simulink model "Balancing_Robot_Nom_Tracking_Quanser"  (R2024b)
settings: Solver=ode23  StartTime=0.0  StopTime=30  RelTol=1e-3
undefined symbols (not defined in the file): C_filter, drv, dspblkCoreblockFVToolHelper, gbox, gcbh, K_Nom_LQR_Br, Nu, Nx, sens, T, wheel
settings Model: Creator=liliy  LastModifiedBy=liliy

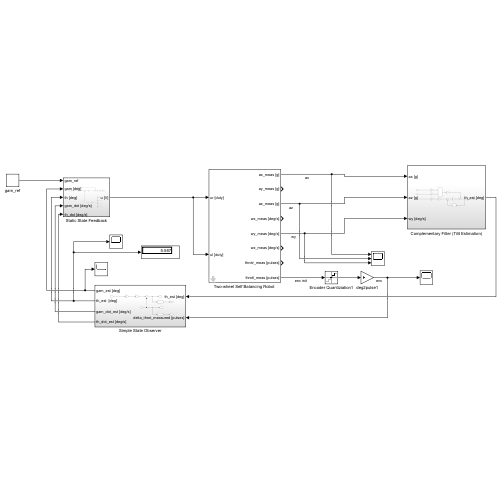
[thumbnail: Simulink's stored preview of the top-level diagram]
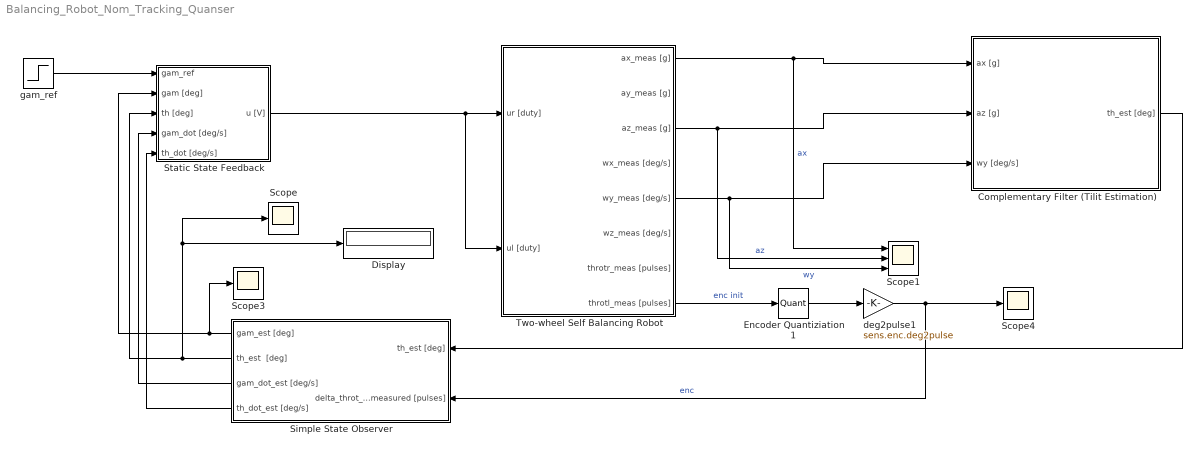
== system Balancing_Robot_Nom_Tracking_Quanser ==
  Complementary Filter (Tilit Estimation) : Subsystem
  Display : Display
  Encoder Quantiziation1 : Quantizer  QuantizationInterval=sens.enc.pulse2deg
  Scope : Scope
  Scope1 : Scope  NumInputPorts=3
  Scope3 : Scope
  Scope4 : Scope
  Simple State Observer : Subsystem
  Static State Feedback : Subsystem
  "Two-wheel Self Balancing Robot " : Subsystem  mask(Balancing robot (longitudinal + lateral dynamics)){initState=[0, 0, 0, 0, 0, 0], Ts=T}
      mask prompts: initState "Initial state [gam(0), psi(0), th(0), dot_gam(0), dot_psi(0), dot_th(0)]'"; Ts "Sample time:"
      mask help:
      | Balancing robot dynamic model.
      | Includes both the longitudinal and lateral (yaw) dynamics.
      mask init:
      | %% General parameters and conversion gains
      | 
      | %   gravity acc [m/s^2]
      | g = 9.81;
      | 
      | %   conversion gains
      | rpm2rads = 2*pi/60;         %   [rpm]   -> [rad/s]
      | rads2rpm = 60/2/pi;         %   [rad/s] -> [rpm]
      | rpm2degs = 360/60;          %   [rpm]   -> [deg/s]
      | degs2rpm = 60/360;          %   [deg/s] -> [rpm]
      | deg2rad = pi/180;           %   [deg]   -> [rad]
      | rad2deg = 180/pi;           %   [rad]   -> [deg]
      | g2ms2 = g;                  %   [acc_g] -> [m/s^2]
      | ms22g = 1/g;                %   [m/s^2] -> [acc_g]
      | ozin2Nm = 0.706e-2;         %   [oz*inch] -> [N*m]
      | 
      | 
      | %%  Battery data
      | 
      | %   electrical data
      | batt.UN = 11.1;     %   nominal voltage
      | 
      | 
      | %%  H-bridge PWM voltage driver
      | 
      | drv.Vbus = batt.UN;                     %   H-bridge DC bus voltage  
      | drv.pwm.bits = 8;                       %   PWM resolution [bits]
      | drv.pwm.levels = 2^drv.pwm.bits;        %   PWM levels
      | drv.pwm.Fs = 490;                       %   PWM frequency
      | drv.dutymax = drv.pwm.levels-1;         %   max duty cycle code
      | drv.duty2V = drv.Vbus/drv.dutymax;      %   duty cycle code (0-255) to voltage
      | drv.V2duty = drv.dutymax/drv.Vbus;      %   voltage to duty cycle code (0-255)
      | 
      | 
      | %%  Gearbox data 
      | 
      | gbox.N = 30;            %   reduction ratio
      | 
      | 
      | %%  Sensors data - Hall-effect encoder
      | 
      | %   Hall-effect encoder
      | sens.enc.ppr = 16*4;    %   pulses per rotation at motor side (w/ quadrature decoding)
      | sens.enc.pulse2deg = 360/sens.enc.ppr;
      | sens.enc.pulse2rad = 2*pi/sens.enc.ppr;
      | sens.enc.deg2pulse = sens.enc.ppr/360;
      | sens.enc.rad2pulse = sens.enc.ppr/2/pi;
      | 
      | 
      | %%  Sensors data - MPU6050 (accelerometer + gyro)
      | 
      | %   center of mass (CoM) position
      | sens.mpu.xb = 0;
      | sens.mpu.yb = 0;
      | sens.mpu.zb = 13.5e-3;
      | 
      | %       MPU6050 embedded accelerometer specs
      | sens.mpu.acc.bits = 16;
      | sens.mpu.acc.fs_g = 16;                                                         %   full-scale in "g" units
      | sens.mpu.acc.fs = sens.mpu.acc.fs_g * g2ms2;                                    %   full-scale in [m/s^2] 
      | sens.mpu.acc.g2LSB = floor(2^(sens.mpu.acc.bits-1)/sens.mpu.acc.fs_g);          %   sensitivity [LSB/g]
      | sens.mpu.acc.ms22LSB = sens.mpu.acc.g2LSB * ms22g;                              %   sensitvity [LSB/(m/s^2)]
      | sens.mpu.acc.LSB2g = sens.mpu.acc.fs_g/2^(sens.mpu.acc.bits-1);                 %   output quantization step [g/LSB]
      | sens.mpu.acc.LSB2ms2 = sens.mpu.acc.LSB2g * g2ms2;                              %   output quantization step [ms2/LSB]
      | sens.mpu.acc.bw = 94;                                                           %   output low-pass filter bandwidth
      | sens.mpu.acc.noisestd = 400e-6*sqrt(100);                                       %   output noise std [g-rms]
      | sens.mpu.acc.noisevar = sens.mpu.acc.noisestd^2;                                %   output noise var [g^2]
      | 
      | %       MPU6050 embdedded gyroscope specs
      | sens.mpu.gyro.bits = 16;
      | sens.mpu.gyro.fs_degs = 250;                                                    %   full scale in [deg/s (dps)]
      | sens.mpu.gyro.fs = sens.mpu.gyro.fs_degs * deg2rad;                             %   full scale in [rad/s]
      | sens.mpu.gyro.degs2LSB = floor(2^(sens.mpu.gyro.bits-1)/sens.mpu.gyro.fs_degs);	%   sensitivity [LSB/degs]
      | sens.mpu.gyro.rads2LSB = sens.mpu.gyro.degs2LSB * rad2deg;                      %   sensitivity [LSB/rads] 
      | sens.mpu.gyro.LSB2degs = sens.mpu.gyro.fs_degs/2^(sens.mpu.gyro.bits-1);        %   output quantization step [degs/LSB]
      | sens.mpu.gyro.LSB2rads = sens.mpu.gyro.LSB2degs * deg2rad;                      %   output quantization step [rads/LSB]
      | sens.mpu.gyro.bw = 98;                                                          %   output low-pass filter bandwidth
      | sens.mpu.gyro.noisestd = 5e-3*sqrt(100);                                        %   output noise std [degs-rms]
      | sens.mpu.gyro.noisevar = sens.mpu.acc.noisestd ^2;                              %   output noise var [degs^2]
      mask Help:
      | Riccardo Antonello (antonello@dei.unipd.it)
      | 
      | May 19, 2020
      | 
      | Dept. of Information Engineering, University of Padova
  deg2pulse1 : Gain  Gain=sens.enc.deg2pulse
  gam_ref : Step  Time=0  After=0.1/wheel.r*rad2deg  SampleTime=0
  wires:
  "Two-wheel Self Balancing Robot "/1(ax_meas [g]) -> Scope1/1, Complementary Filter (Tilit Estimation)/1(ax [g])  "ax"
  "Two-wheel Self Balancing Robot "/3(az_meas [g]) -> Scope1/2, Complementary Filter (Tilit Estimation)/2(az [g])  "az"
  "Two-wheel Self Balancing Robot "/5(wy_meas [deg/s]) -> Scope1/3, Complementary Filter (Tilit Estimation)/3(wy [deg/s])  "wy"
  Complementary Filter (Tilit Estimation)/1(th_est [deg]) -> Simple State Observer/1(th_est [deg])
  Simple State Observer/1(gam_est [deg]) -> Scope3/1, Static State Feedback/2(gam [deg])
  Simple State Observer/2(th_est  [deg]) -> Scope/1, Display/1, Static State Feedback/3(th [deg])
  Simple State Observer/3(gam_dot_est [deg/s]) -> Static State Feedback/4(gam_dot [deg/s])
  Simple State Observer/4(th_dot_est [deg/s]) -> Static State Feedback/5(th_dot [deg/s])
  gam_ref/1 -> Static State Feedback/1(gam_ref)
  Static State Feedback/1(u [V]) -> "Two-wheel Self Balancing Robot "/2(ul [duty]), "Two-wheel Self Balancing Robot "/1(ur [duty])
  Encoder Quantiziation1/1 -> deg2pulse1/1
  "Two-wheel Self Balancing Robot "/8(throtl_meas [pulses]) -> Encoder Quantiziation1/1  "enc init"
  deg2pulse1/1 -> Scope4/1, Simple State Observer/2(delta_throt_measured [pulses])  "enc"

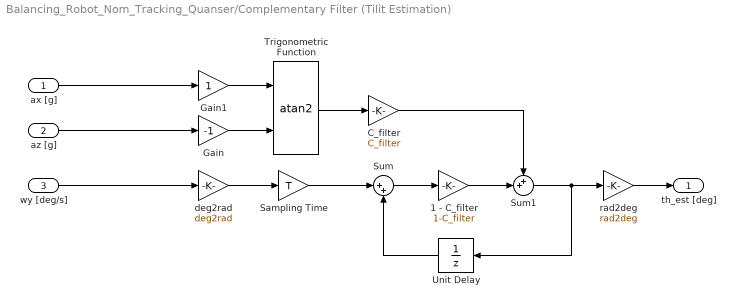
== system Balancing_Robot_Nom_Tracking_Quanser/Complementary Filter (Tilit Estimation) ==
  ax [g] : Inport
  az [g] : Inport  Port=2
  wy [deg/s] : Inport  Port=3
  1 - C_filter : Gain  Gain=1-C_filter
  C_filter : Gain  Gain=C_filter
  Gain : Gain  Gain=-1
  Gain1 : Gain
  Sampling Time : Gain  Gain=T
  Sum : Sum  Inputs=|++
  Sum1 : Sum  Inputs=++|
  Trigonometric Function : Trigonometry  Operator=atan2
  Unit Delay : UnitDelay  SampleTime=T  HasFrameUpgradeWarning=on
  deg2rad : Gain  Gain=deg2rad
  rad2deg : Gain  Gain=rad2deg
  th_est [deg] : Outport
  wires:
  Trigonometric Function/1 -> C_filter/1
  Gain/1 -> Trigonometric Function/2
  rad2deg/1 -> th_est [deg]/1
  deg2rad/1 -> Sampling Time/1
  Sum/1 -> 1 - C_filter/1
  Gain1/1 -> Trigonometric Function/1
  Sum1/1 -> Unit Delay/1, rad2deg/1
  Sampling Time/1 -> Sum/1
  1 - C_filter/1 -> Sum1/2
  Unit Delay/1 -> Sum/2
  C_filter/1 -> Sum1/1
  ax [g]/1 -> Gain1/1
  az [g]/1 -> Gain/1
  wy [deg/s]/1 -> deg2rad/1

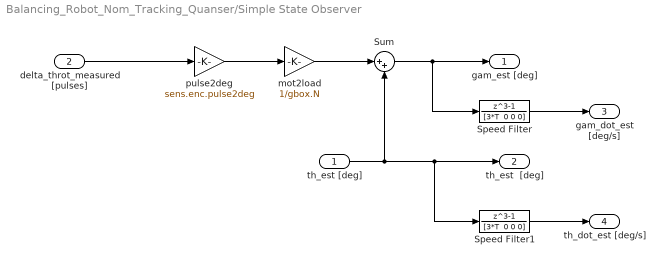
== system Balancing_Robot_Nom_Tracking_Quanser/Simple State Observer ==
  th_est [deg] : Inport
  delta_throt_measured [pulses] : Inport  Port=2
  Speed Filter : DiscreteTransferFcn  LoadFcn=dspblkCoreblockFVToolHelper(gcbh,'load');  Numerator=[1 0 0 -1]  Denominator="[3*T  0 0 0]"
      settings: CopyFcn=dspblkCoreblockFVToolHelper(gcbh,'copy');  DeleteFcn=dspblkCoreblockFVToolHelper(gcbh,'close');  ModelCloseFcn=dspblkCoreblockFVToolHelper(gcbh,'close');  PreSaveFcn=dspblkCoreblockFVToolHelper(gcbh,'presave');  PostSaveFcn=dspblkCoreblockFVToolHelper(gcbh,'postsave');  CloseFcn=dspblkCoreblockFVToolHelper(gcbh,'close');
  Speed Filter1 : DiscreteTransferFcn  LoadFcn=dspblkCoreblockFVToolHelper(gcbh,'load');  Numerator=[1 0 0 -1]  Denominator="[3*T  0 0 0]"
      settings: CopyFcn=dspblkCoreblockFVToolHelper(gcbh,'copy');  DeleteFcn=dspblkCoreblockFVToolHelper(gcbh,'close');  ModelCloseFcn=dspblkCoreblockFVToolHelper(gcbh,'close');  PreSaveFcn=dspblkCoreblockFVToolHelper(gcbh,'presave');  PostSaveFcn=dspblkCoreblockFVToolHelper(gcbh,'postsave');  CloseFcn=dspblkCoreblockFVToolHelper(gcbh,'close');
  Sum : Sum  Inputs=|++
  mot2load : Gain  Gain=1/gbox.N
  pulse2deg : Gain  Gain=sens.enc.pulse2deg
  gam_est [deg] : Outport
  th_est  [deg] : Outport  Port=2
  gam_dot_est [deg/s] : Outport  Port=3
  th_dot_est [deg/s] : Outport  Port=4
  wires:
  Sum/1 -> Speed Filter/1, gam_est [deg]/1
  pulse2deg/1 -> mot2load/1
  Speed Filter/1 -> gam_dot_est [deg/s]/1
  delta_throt_measured [pulses]/1 -> pulse2deg/1
  Speed Filter1/1 -> th_dot_est [deg/s]/1
  th_est [deg]/1 -> Sum/2, Speed Filter1/1, th_est  [deg]/1
  mot2load/1 -> Sum/1

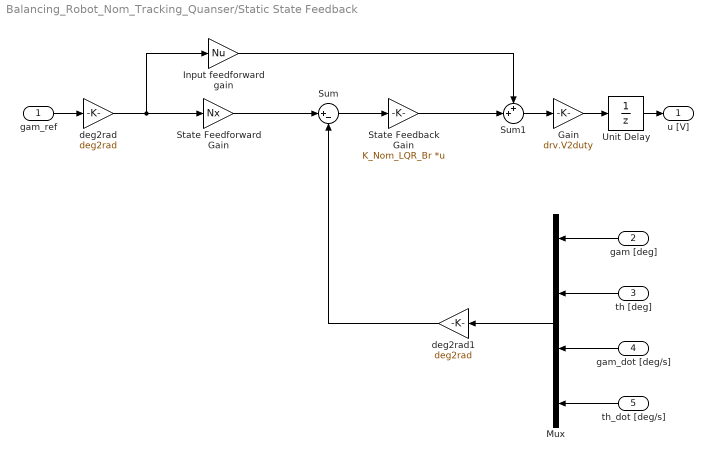
== system Balancing_Robot_Nom_Tracking_Quanser/Static State Feedback ==
  gam_ref : Inport
  gam [deg] : Inport  Port=2
  th [deg] : Inport  Port=3
  gam_dot [deg/s] : Inport  Port=4
  th_dot [deg/s] : Inport  Port=5
  Gain : Gain  Gain=drv.V2duty
  Input feedforward gain : Gain  Gain=Nu
  Mux : Mux
  State Feedback Gain : Gain  Gain=K_Nom_LQR_Br  Multiplication=Matrix(K*u)
  State Feedforward Gain : Gain  Gain=Nx
  Sum : Sum  Inputs=|+-
  Sum1 : Sum  Inputs=++|
  Unit Delay : UnitDelay  SampleTime=T  HasFrameUpgradeWarning=on
  deg2rad : Gain  Gain=deg2rad
  deg2rad1 : Gain  Gain=deg2rad
  u [V] : Outport
  wires:
  gam_ref/1 -> deg2rad/1
  deg2rad/1 -> Input feedforward gain/1, State Feedforward Gain/1
  State Feedforward Gain/1 -> Sum/1
  Sum/1 -> State Feedback Gain/1
  State Feedback Gain/1 -> Sum1/2
  Input feedforward gain/1 -> Sum1/1
  Sum1/1 -> Gain/1
  Mux/1 -> deg2rad1/1
  gam_dot [deg/s]/1 -> Mux/3
  th_dot [deg/s]/1 -> Mux/4
  Gain/1 -> Unit Delay/1
  gam [deg]/1 -> Mux/1
  th [deg]/1 -> Mux/2
  deg2rad1/1 -> Sum/2
  Unit Delay/1 -> u [V]/1

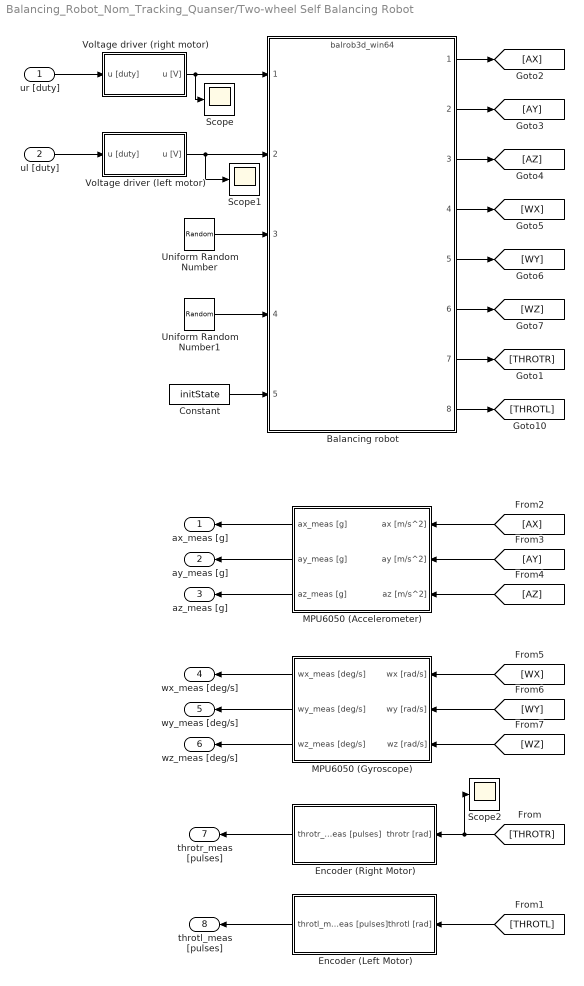
== system Balancing_Robot_Nom_Tracking_Quanser/Two-wheel Self Balancing Robot  ==
  ur [duty] : Inport
  ul [duty] : Inport  Port=2
  Balancing robot : ModelReference  ModelNameDialog=balrob3d_win64.slxp  ModelReferenceVersion=1.741  CopyOfModelProtected=on
  Constant : Constant  Value=initState
  Encoder (Left Motor) : Subsystem
  Encoder (Right Motor) : Subsystem
  MPU6050 (Accelerometer) : Subsystem
  MPU6050 (Gyroscope) : Subsystem
  Scope : Scope
  Scope1 : Scope
  Scope2 : Scope
  Uniform Random Number : UniformRandomNumber  Minimum=0.7  Maximum=1.3  SampleTime=1
  Uniform Random Number1 : UniformRandomNumber  Minimum=0.7  Maximum=1.3  Seed=10  SampleTime=1
  Voltage driver (left motor) : Subsystem
  Voltage driver (right motor) : Subsystem
  ax_meas [g] : Outport
  ay_meas [g] : Outport  Port=2
  az_meas [g] : Outport  Port=3
  wx_meas [deg/s] : Outport  Port=4
  wy_meas [deg/s] : Outport  Port=5
  wz_meas [deg/s] : Outport  Port=6
  throtr_meas [pulses] : Outport  Port=7
  throtl_meas [pulses] : Outport  Port=8
  wires:
  ur [duty]/1 -> Voltage driver (right motor)/1(u [duty])
  [WX] -> MPU6050 (Gyroscope)/1(wx [rad/s])
  Balancing robot/2 -> [AY]
  Balancing robot/4 -> [WX]
  Balancing robot/8 -> [THROTL]
  Balancing robot/1 -> [AX]
  [THROTL] -> Encoder (Left Motor)/1(throtl [rad])
  Balancing robot/6 -> [WZ]
  Balancing robot/7 -> [THROTR]
  Balancing robot/5 -> [WY]
  [AX] -> MPU6050 (Accelerometer)/1(ax [m/s^2])
  [WY] -> MPU6050 (Gyroscope)/2(wy [rad/s])
  Balancing robot/3 -> [AZ]
  [WZ] -> MPU6050 (Gyroscope)/3(wz [rad/s])
  [AZ] -> MPU6050 (Accelerometer)/3(az [m/s^2])
  [THROTR] -> Scope2/1, Encoder (Right Motor)/1(throtr [rad])
  ul [duty]/1 -> Voltage driver (left motor)/1(u [duty])
  [AY] -> MPU6050 (Accelerometer)/2(ay [m/s^2])
  MPU6050 (Accelerometer)/1(ax_meas [g]) -> ax_meas [g]/1
  MPU6050 (Accelerometer)/2(ay_meas [g]) -> ay_meas [g]/1
  MPU6050 (Accelerometer)/3(az_meas [g]) -> az_meas [g]/1
  MPU6050 (Gyroscope)/1(wx_meas [deg/s]) -> wx_meas [deg/s]/1
  MPU6050 (Gyroscope)/2(wy_meas [deg/s]) -> wy_meas [deg/s]/1
  MPU6050 (Gyroscope)/3(wz_meas [deg/s]) -> wz_meas [deg/s]/1
  Encoder (Right Motor)/1(throtr_meas [pulses]) -> throtr_meas [pulses]/1
  Encoder (Left Motor)/1(throtl_meas [pulses]) -> throtl_meas [pulses]/1
  Voltage driver (right motor)/1(u [V]) -> Scope/1, Balancing robot/1
  Voltage driver (left motor)/1(u [V]) -> Scope1/1, Balancing robot/2
  Uniform Random Number/1 -> Balancing robot/3
  Uniform Random Number1/1 -> Balancing robot/4
  Constant/1 -> Balancing robot/5

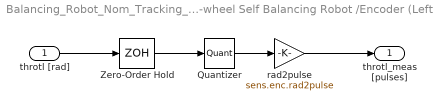
== system Balancing_Robot_Nom_Tracking_Quanser/Two-wheel Self Balancing Robot /Encoder (Left Motor) ==
  throtl [rad] : Inport
  Quantizer : Quantizer  QuantizationInterval=sens.enc.pulse2rad
  Zero-Order Hold : ZeroOrderHold  SampleTime=Ts
  rad2pulse : Gain  Gain=sens.enc.rad2pulse
  throtl_meas [pulses] : Outport
  wires:
  Quantizer/1 -> rad2pulse/1
  Zero-Order Hold/1 -> Quantizer/1
  throtl [rad]/1 -> Zero-Order Hold/1
  rad2pulse/1 -> throtl_meas [pulses]/1

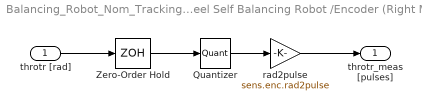
== system Balancing_Robot_Nom_Tracking_Quanser/Two-wheel Self Balancing Robot /Encoder (Right Motor) ==
  throtr [rad] : Inport
  Quantizer : Quantizer  QuantizationInterval=sens.enc.pulse2rad
  Zero-Order Hold : ZeroOrderHold  SampleTime=Ts
  rad2pulse : Gain  Gain=sens.enc.rad2pulse
  throtr_meas [pulses] : Outport
  wires:
  throtr [rad]/1 -> Zero-Order Hold/1
  Zero-Order Hold/1 -> Quantizer/1
  Quantizer/1 -> rad2pulse/1
  rad2pulse/1 -> throtr_meas [pulses]/1

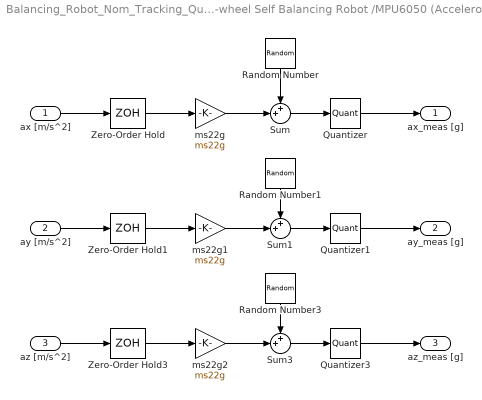
== system Balancing_Robot_Nom_Tracking_Quanser/Two-wheel Self Balancing Robot /MPU6050 (Accelerometer) ==
  ax [m/s^2] : Inport
  ay [m/s^2] : Inport  Port=2
  az [m/s^2] : Inport  Port=3
  Quantizer : Quantizer  QuantizationInterval=sens.mpu.acc.LSB2g
  Quantizer1 : Quantizer  QuantizationInterval=sens.mpu.acc.LSB2g
  Quantizer3 : Quantizer  QuantizationInterval=sens.mpu.acc.LSB2g
  Random Number : RandomNumber  Variance=sens.mpu.acc.noisevar  Seed=1  SampleTime=Ts
  Random Number1 : RandomNumber  Variance=sens.mpu.acc.noisevar  Seed=10  SampleTime=Ts
  Random Number3 : RandomNumber  Variance=sens.mpu.acc.noisevar  Seed=100  SampleTime=Ts
  Sum : Sum  Inputs=++|
  Sum1 : Sum  Inputs=++|
  Sum3 : Sum  Inputs=++|
  Zero-Order Hold : ZeroOrderHold  SampleTime=Ts
  Zero-Order Hold1 : ZeroOrderHold  SampleTime=Ts
  Zero-Order Hold3 : ZeroOrderHold  SampleTime=Ts
  ms22g : Gain  Gain=ms22g
  ms22g1 : Gain  Gain=ms22g
  ms22g2 : Gain  Gain=ms22g
  ax_meas [g] : Outport
  ay_meas [g] : Outport  Port=2
  az_meas [g] : Outport  Port=3
  wires:
  ax [m/s^2]/1 -> Zero-Order Hold/1
  Zero-Order Hold1/1 -> ms22g1/1
  Sum1/1 -> Quantizer1/1
  ms22g/1 -> Sum/2
  ay [m/s^2]/1 -> Zero-Order Hold1/1
  Sum3/1 -> Quantizer3/1
  ms22g1/1 -> Sum1/2
  Random Number1/1 -> Sum1/1
  Random Number/1 -> Sum/1
  Sum/1 -> Quantizer/1
  Random Number3/1 -> Sum3/1
  ms22g2/1 -> Sum3/2
  Zero-Order Hold3/1 -> ms22g2/1
  az [m/s^2]/1 -> Zero-Order Hold3/1
  Zero-Order Hold/1 -> ms22g/1
  Quantizer/1 -> ax_meas [g]/1
  Quantizer1/1 -> ay_meas [g]/1
  Quantizer3/1 -> az_meas [g]/1

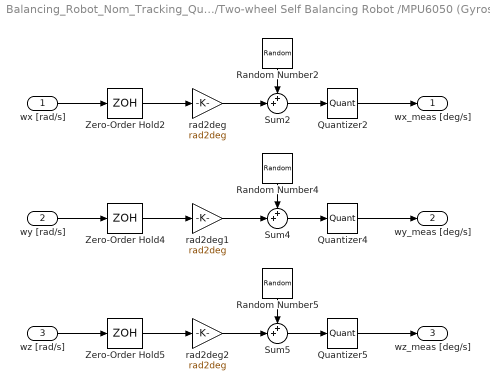
== system Balancing_Robot_Nom_Tracking_Quanser/Two-wheel Self Balancing Robot /MPU6050 (Gyroscope) ==
  wx [rad/s] : Inport
  wy [rad/s] : Inport  Port=2
  wz [rad/s] : Inport  Port=3
  Quantizer2 : Quantizer  QuantizationInterval=sens.mpu.gyro.LSB2degs
  Quantizer4 : Quantizer  QuantizationInterval=sens.mpu.gyro.LSB2degs
  Quantizer5 : Quantizer  QuantizationInterval=sens.mpu.gyro.LSB2degs
  Random Number2 : RandomNumber  Variance=sens.mpu.gyro.noisevar  Seed=2  SampleTime=Ts
  Random Number4 : RandomNumber  Variance=sens.mpu.gyro.noisevar  Seed=20  SampleTime=Ts
  Random Number5 : RandomNumber  Variance=sens.mpu.gyro.noisevar  Seed=200  SampleTime=Ts
  Sum2 : Sum  Inputs=++|
  Sum4 : Sum  Inputs=++|
  Sum5 : Sum  Inputs=++|
  Zero-Order Hold2 : ZeroOrderHold  SampleTime=Ts
  Zero-Order Hold4 : ZeroOrderHold  SampleTime=Ts
  Zero-Order Hold5 : ZeroOrderHold  SampleTime=Ts
  rad2deg : Gain  Gain=rad2deg
  rad2deg1 : Gain  Gain=rad2deg
  rad2deg2 : Gain  Gain=rad2deg
  wx_meas [deg/s] : Outport
  wy_meas [deg/s] : Outport  Port=2
  wz_meas [deg/s] : Outport  Port=3
  wires:
  Random Number2/1 -> Sum2/1
  Sum2/1 -> Quantizer2/1
  Quantizer2/1 -> wx_meas [deg/s]/1
  Zero-Order Hold5/1 -> rad2deg2/1
  Sum4/1 -> Quantizer4/1
  rad2deg/1 -> Sum2/2
  rad2deg2/1 -> Sum5/2
  Random Number5/1 -> Sum5/1
  Zero-Order Hold4/1 -> rad2deg1/1
  Sum5/1 -> Quantizer5/1
  Random Number4/1 -> Sum4/1
  Zero-Order Hold2/1 -> rad2deg/1
  Quantizer5/1 -> wz_meas [deg/s]/1
  wz [rad/s]/1 -> Zero-Order Hold5/1
  wx [rad/s]/1 -> Zero-Order Hold2/1
  rad2deg1/1 -> Sum4/2
  Quantizer4/1 -> wy_meas [deg/s]/1
  wy [rad/s]/1 -> Zero-Order Hold4/1

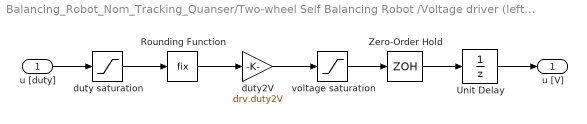
== system Balancing_Robot_Nom_Tracking_Quanser/Two-wheel Self Balancing Robot /Voltage driver (left motor) ==
  u [duty] : Inport
  Rounding Function : Rounding  Operator=fix
  Unit Delay : UnitDelay  SampleTime=1/drv.pwm.Fs  HasFrameUpgradeWarning=on
  Zero-Order Hold : ZeroOrderHold  SampleTime=Ts
  duty saturation : Saturate  UpperLimit=255  LowerLimit=-255
  duty2V : Gain  Gain=drv.duty2V
  voltage saturation : Saturate  UpperLimit=drv.Vbus  LowerLimit=-drv.Vbus
  u [V] : Outport
  wires:
  Zero-Order Hold/1 -> Unit Delay/1
  u [duty]/1 -> duty saturation/1
  voltage saturation/1 -> Zero-Order Hold/1
  duty saturation/1 -> Rounding Function/1
  Rounding Function/1 -> duty2V/1
  duty2V/1 -> voltage saturation/1
  Unit Delay/1 -> u [V]/1

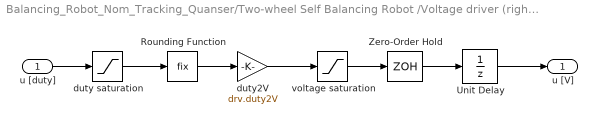
== system Balancing_Robot_Nom_Tracking_Quanser/Two-wheel Self Balancing Robot /Voltage driver (right motor) ==
  u [duty] : Inport
  Rounding Function : Rounding  Operator=fix
  Unit Delay : UnitDelay  SampleTime=1/drv.pwm.Fs  HasFrameUpgradeWarning=on
  Zero-Order Hold : ZeroOrderHold  SampleTime=Ts
  duty saturation : Saturate  UpperLimit=255  LowerLimit=-255
  duty2V : Gain  Gain=drv.duty2V
  voltage saturation : Saturate  UpperLimit=drv.Vbus  LowerLimit=-drv.Vbus
  u [V] : Outport
  wires:
  u [duty]/1 -> duty saturation/1
  duty saturation/1 -> Rounding Function/1
  Zero-Order Hold/1 -> Unit Delay/1
  voltage saturation/1 -> Zero-Order Hold/1
  Rounding Function/1 -> duty2V/1
  duty2V/1 -> voltage saturation/1
  Unit Delay/1 -> u [V]/1
